simulink model "model"  (R2025a)
settings: Solver=VariableStepAuto  StartTime=0.0  StopTime=10.0  RelTol=1e-3
undefined symbols (not defined in the file): g, I_zz, L_cg, m
libraries: simulink_extras x1
settings Model: Creator=akshat  LastModifiedBy=akshat

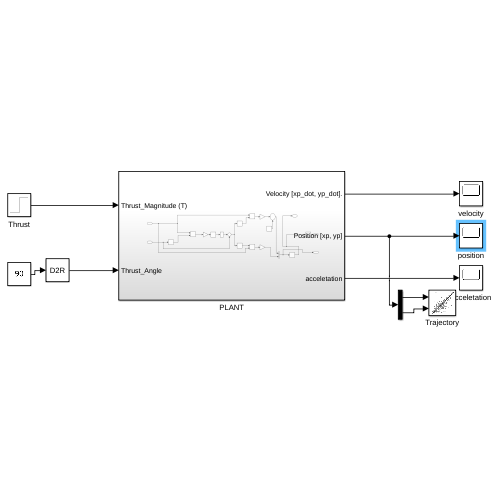
[thumbnail: Simulink's stored preview of the top-level diagram]
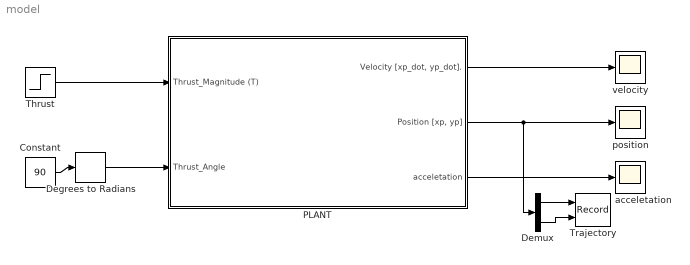
== system model ==
  Constant : Constant  Value=90
  Degrees to Radians : simulink_extras/Transformations/Degrees to Radians
  Demux : Demux  Outputs=2
  PLANT : Subsystem
  Thrust : Step  After=30  SampleTime=0
  Trajectory : Record  NumPorts=2.0  FileSettingsInternal="{\"entries\":[{\"content\":{\"excelSettings\":{\"content\":{},\"type\":\"Streamout.ExcelSettings\"},\"parquetSettings\":{\"content\":{},\"type\":\"Streamout.ParquetSettings\"}},\"type\":\"Streamout.FileSettingStorage\",\"uuid\":\"\"}],\"packageUris\":[\"http:\\/\\/schema.mathworks.com\\/mf0\\/streamout_blocks\\/R2020a\"],\"version\":\"1.0\"}"  FrameSettings=[0, 0]  Layout=[1 1]  SignalsInternal="{\"entries\":[{\"content\":{\"signals\":[{\"content\":{\"blockPath\":[],\"dimensions\":[1],\"domain\":\"\",\"lineColor\":\"#edb120\",\"lineWidth\":2,\"plots\":[ 1 ],\"port\":1,\"sid\":[\"\"],\"signalID\":1,\"signalName\":\"Demux:1\"},\"type\":\"RecordBlkView.Signal\",\"uuid\":\"\"},{\"content\":{\"blockPath\":[],\"dimensions\":[1],\"domain\":\"\",\"lineColor\":\"#7e2f8e\",\"lineWidth\":2,\"plots\":[ 1 ],\"port\":2,\"sid\":[\"\"],\"signalID\":2,\"signalName\":\"Demux:2\"},\"type\":\"RecordBlkView.Signal\",\"uuid\":\"\"}]},\"type\":\"RecordBlkView.InputSignals\",\"uuid\":\"\"}],\"packageUris\":[\"http:\\/\\/schema.mathworks.com\\/mf0\\/streamout_blocks\\/R2020a\"],\"version\":\"1.0\"}"  VisualizationBindings="{\"xyplotplugin\":{\"info\":[{\"series\":[{\"bindingParametersList\":[{\"parameter\":\"X-Axis\",\"signalID\":1,\"signalName\":\"Demux:1\"},{\"parameter\":\"Y-Axis\",\"signalID\":2,\"signalName\":\"Demux:2\"}],\"seriesID\":0}],\"subplotID\":1}]}}"  CompatibilityTag=XY
  acceletation : Scope
      settings: ActiveDisplayYMinimum=-1  ActiveDisplayYMaximum=1  DataLoggingVariableName=ScopeData2
  position : Scope
      settings: ActiveDisplayYMinimum=-547.26744355774088  ActiveDisplayYMaximum=60.807493728637866
  velocity : Scope
      settings: ActiveDisplayYMinimum=-1  ActiveDisplayYMaximum=1
  wires:
  PLANT/1("Velocity [xp_dot, yp_dot].") -> velocity/1
  PLANT/2("Position [xp, yp]") -> Demux/1, position/1
  PLANT/3(acceletation) -> acceletation/1
  Thrust/1 -> PLANT/1(Thrust_Magnitude (T))
  Degrees to Radians/1 -> PLANT/2(Thrust_Angle)
  Constant/1 -> Degrees to Radians/1
  Demux/1 -> Trajectory/1
  Demux/2 -> Trajectory/2

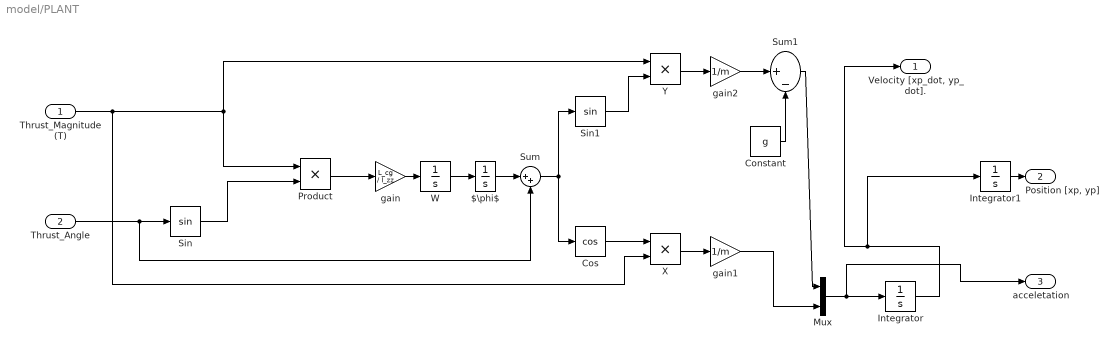
== system model/PLANT ==
  Thrust_Magnitude (T) : Inport
  Thrust_Angle : Inport  Port=2
  $\phi$ : Integrator
  Constant : Constant  Value=g
  Cos : Trigonometry  Operator=cos
  Integrator : Integrator
  Integrator1 : Integrator
  Mux : Mux  Inputs=2
  Product : Product
  Sin : Trigonometry
  Sin1 : Trigonometry
  Sum : Sum  Inputs=|++
  Sum1 : Sum  Inputs=|+-
  W : Integrator
  X : Product
  Y : Product
  gain : Gain  Gain=L_cg / I_zz
  gain1 : Gain  Gain=1/m
  gain2 : Gain  Gain=1/m
  "Velocity [xp_dot, yp_dot]." : Outport
  "Position [xp, yp]" : Outport  Port=2
  acceletation : Outport  Port=3
  wires:
  Thrust_Angle/1 -> Sin/1, Sum/2
  Sin/1 -> Product/2
  Product/1 -> gain/1
  gain/1 -> W/1
  W/1 -> $\phi$/1
  $\phi$/1 -> Sum/1
  Sum/1 -> Cos/1, Sin1/1
  Sin1/1 -> Y/2
  Cos/1 -> X/1
  Thrust_Magnitude (T)/1 -> X/2, Y/1, Product/1
  X/1 -> gain1/1
  Y/1 -> gain2/1
  Sum1/1 -> Mux/1
  gain2/1 -> Sum1/1
  Constant/1 -> Sum1/2
  Mux/1 -> acceletation/1, Integrator/1
  gain1/1 -> Mux/2
  Integrator/1 -> Integrator1/1, "Velocity [xp_dot, yp_dot]."/1
  Integrator1/1 -> "Position [xp, yp]"/1
